simulink model "ScissorLift_Simulink_Multibody"  (R2026a)
settings: Solver=ode15s  StopTime=5  MaxStep=0.01  RelTol=1e-6  AbsTol=1e-8
PostLoadFcn:
  | addpath(fullfile(fileparts(get_param(bdroot,'FileName')),'Geometry'));
model workspace (MAT data in the model file):
  density_kg_m3 = 7850
undefined symbols (not defined in the file): X, Y, Z
libraries: sm_lib x69, nesl_utility x2
(part 2 of 2)

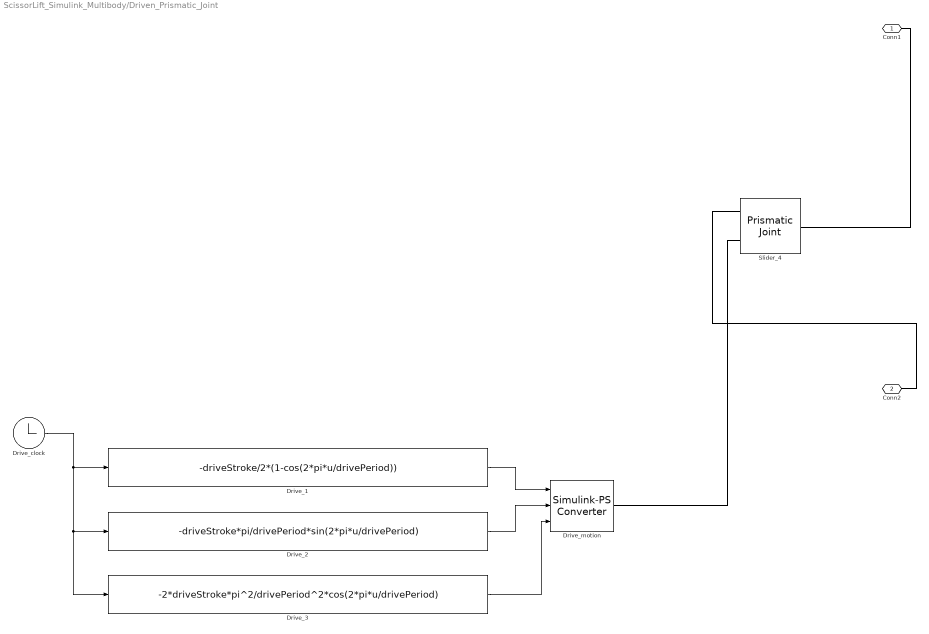
== system ScissorLift_Simulink_Multibody/Driven_Prismatic_Joint ==
  Drive_1 : Fcn  Expr=-driveStroke/2*(1-cos(2*pi*u/drivePeriod))
  Drive_2 : Fcn  Expr=-driveStroke*pi/drivePeriod*sin(2*pi*u/drivePeriod)
  Drive_3 : Fcn  Expr=-2*driveStroke*pi^2/drivePeriod^2*cos(2*pi*u/drivePeriod)
  Drive_clock : Clock
  Drive_motion : nesl_utility/Simulink-PS Converter  PhysicalDomain=network_engine_domain  SubClassName=ps_input  LeftPortType=input  RightPortType=output  PseudoPeriodic=off  Frequencies=[]  NoiseDistribution=none  NoiseParameters=[]  Unit=m  AffineConversion=off  FilteringAndDerivatives=provide  SimscapeFilterOrder=1  InputFilterTimeConstant=0.001  UdotUserProvided=2
  Slider_4 : sm_lib/Joints/Prismatic Joint  JointMode=Normal  CompositeWrenchDir=FollowerOnBase  CompositeWrenchFrame=BaseFrame  SenseConstraintForce=off  SenseConstraintTorque=off  SenseTotalForce=off  SenseTotalTorque=off  PositionTargetSpecify=off  PositionTargetPriority=High  PositionTargetValue=0  PositionTargetValueUnits=m  VelocityTargetSpecify=off  VelocityTargetPriority=High  VelocityTargetValue=0  VelocityTargetValueUnits=m/s  EquilibriumPosition=0  EquilibriumPositionUnits=m  SpringStiffness=0  SpringStiffnessUnits=N/m  DampingCoefficient=0  DampingCoefficientUnits=N/(m/s)  LowerLimitSpecify=on  LowerLimitBound=-0.023  LowerLimitBoundUnits=m  LowerLimitStiffness=1e6  LowerLimitStiffnessUnits=N/m  LowerLimitDamping=1e3  LowerLimitDampingUnits=N/(m/s)  LowerLimitTransitionRegionWidth=1e-4  LowerLimitTransitionRegionWidthUnits=m  UpperLimitSpecify=on  UpperLimitBound=0  UpperLimitBoundUnits=m  UpperLimitStiffness=1e6  UpperLimitStiffnessUnits=N/m  UpperLimitDamping=1e3  UpperLimitDampingUnits=N/(m/s)  UpperLimitTransitionRegionWidth=1e-4  UpperLimitTransitionRegionWidthUnits=m  TorqueActuationMode=ComputedTorque  MotionActuationMode=InputMotion  SensePosition=off  SenseVelocity=off  SenseAcceleration=off  SenseTorqueForce=off  SenseLowerLimitTorqueForce=off  SenseUpperLimitTorqueForce=off
  Conn1 : PMIOPort  Side=Right
  Conn2 : PMIOPort  Port=2  Side=Left
  wires:
  Drive_3/1 -> Drive_motion/3
  Drive_clock/1 -> Drive_2/1, Drive_3/1, Drive_1/1
  Drive_1/1 -> Drive_motion/1
  Drive_2/1 -> Drive_motion/2
  connections:
  Conn2/RConn1 -- Slider_4/LConn1
  Drive_motion/RConn1 -- Slider_4/LConn2
  Slider_4/RConn1 -- Conn1/RConn1
